simulink model "Sensors"  (R2026b)
settings: Solver=VariableStepAuto
settings Model: Creator=Dani  LastModifiedBy=Dani

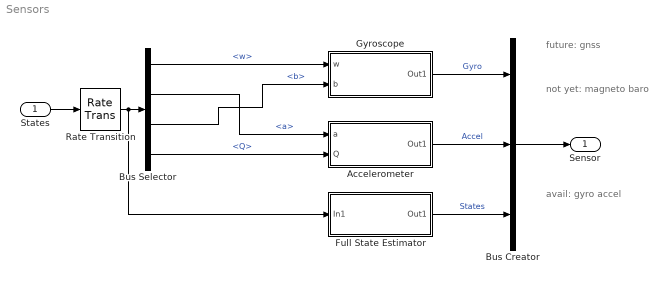
== system Sensors ==
  note: future:
      | gnss
  note: not yet:
      | magneto
      | baro
  note: avail:
      | gyro
      | accel
  States : Inport
  Accelerometer : Subsystem
  Bus Creator : BusCreator  Inputs=3
  Bus Selector : BusSelector  OutputSignals=w,a,b,Q
  Full State Estimator : Subsystem
  Gyroscope : Subsystem
  Rate Transition : RateTransition
  Sensor : Outport
  wires:
  States/1 -> Rate Transition/1
  Rate Transition/1 -> Bus Selector/1, Full State Estimator/1(In1)
  Bus Selector/4 -> Accelerometer/2(Q)  "<Q>"
  Bus Selector/3 -> Gyroscope/2(b)  "<b>"
  Bus Selector/2 -> Accelerometer/1(a)  "<a>"
  Bus Selector/1 -> Gyroscope/1(w)  "<w>"
  Gyroscope/1(Out1) -> Bus Creator/1  "Gyro"
  Accelerometer/1(Out1) -> Bus Creator/2  "Accel"
  Bus Creator/1 -> Sensor/1
  Full State Estimator/1(Out1) -> Bus Creator/3  "States"

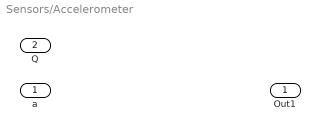
== system Sensors/Accelerometer ==
  a : Inport
  Q : Inport  Port=2
  Out1 : Outport
  wires:
  ? -> Out1/1

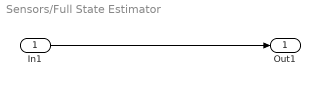
== system Sensors/Full State Estimator ==
  In1 : Inport
  Out1 : Outport
  wires:
  In1/1 -> Out1/1

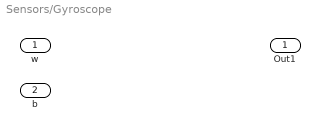
== system Sensors/Gyroscope ==
  w : Inport
  b : Inport  Port=2
  Out1 : Outport
